simulink model "Simulation_cs_old"  (R2019a)
settings: Solver=ode5  StartTime=0.0  StopTime=inf  FixedStep=1/20  RelTol=1e-3
PreLoadFcn:
  | mbxruntime.callbacks.PreLoadFcn(bdroot);
PostLoadFcn:
  | mbxruntime.callbacks.PostLoadFcn(bdroot);
InitFcn:
  | mbxruntime.callbacks.InitFcn(bdroot);
StartFcn:
  | mbxruntime.callbacks.StartFcn(bdroot);
StopFcn:
  | mbxruntime.callbacks.StopFcn(bdroot);
model workspace: external: MAT-File .\Simulation_cs_hws.mat (data not in the file)
undefined symbols (not defined in the file or in its folder): DiscIntNeverNeededParam, InitImageOutputDir, mbxruntime, Simulation_cs_3ba1e87c6cdc7fd9, Simulation_cs_BMW_X5_SUV_1_Dynamics_Empty_STATE_BMW_X5_SUV_1_x0, Simulation_cs_BMW_X5_SUV_1_Dynamics_Empty_STATE_BMW_X5_SUV_1_y0, Simulation_cs_BMW_X5_SUV_1_Dynamics_Empty_STATE_BMW_X5_SUV_1_z0, Simulation_cs_dbe7801ee2d75073, Simulation_cs_f34d2d8469e03015
libraries: adeye_lib x45, robotlib x3, PreScanSimulinkLibrary x2, PreScanUsefulBlocks x1
(part 2 of 3)

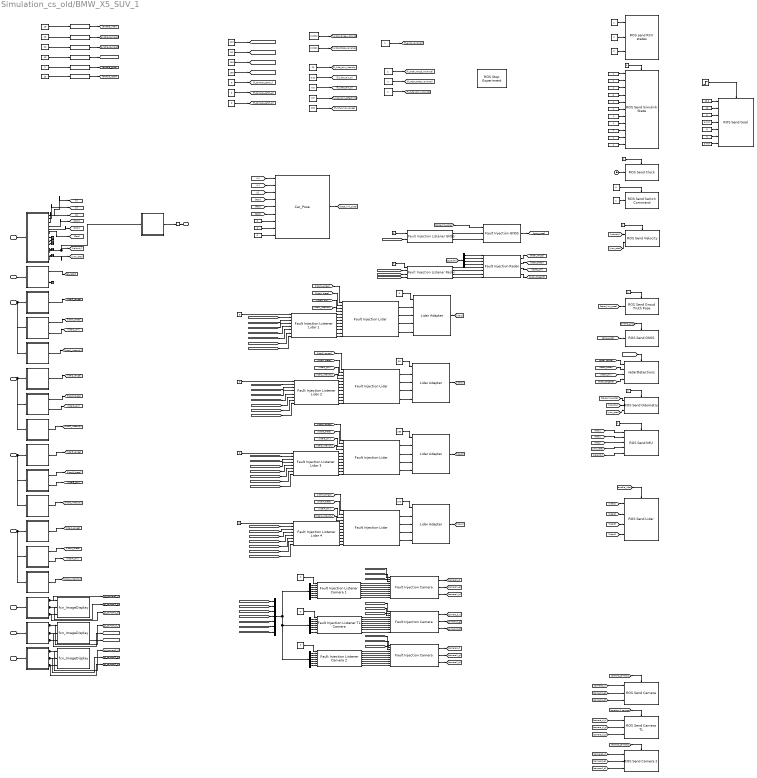
== system Simulation_cs_old/BMW_X5_SUV_1 ==
  note: CoG  compared
      | to the backwheels
      | center
  note: Lidar Fault injection Constants
  note: Radar Fault Injection Constants
  note: Rain model, Constants
  note: Camera Fault injection Constants
  note: GNSS Fault Injection Constants
  note: Gaussian random noise, Parameters
  note: Patch
  note: Frequencies at which the messages are sent
      |
      | For this send frequency to be respected, the simulink compilation sheet frequency
      | needs to be an integer multiple of this send frequency.
  SELF_BMW_X5_SUV_1 : Inport  Tag=inport/SelfPort  OutDataTypeStr=Bus: PRESCAN_SELFSENSORDATA  PortDimensions=1  SampleTime=1/20  BusOutputAsStruct=on
  Radar_1 : Inport  Tag=inport/Radar  Port=2  OutDataTypeStr=Bus: PRESCAN_SCANNERSENSOR_MESSAGE  PortDimensions=7  SampleTime=1/20  BusOutputAsStruct=on
  PointCloudSensor_1 : Inport  Tag=inport/PointCloudInport  Port=3  OutDataTypeStr=single  SampleTime=1/20  BusOutputAsStruct=on
  PointCloudSensor_2 : Inport  Tag=inport/PointCloudInport  Port=4  OutDataTypeStr=single  SampleTime=1/20  BusOutputAsStruct=on
  PointCloudSensor_3 : Inport  Tag=inport/PointCloudInport  Port=5  OutDataTypeStr=single  SampleTime=1/20  BusOutputAsStruct=on
  PointCloudSensor_4 : Inport  Tag=inport/PointCloudInport  Port=6  OutDataTypeStr=single  SampleTime=1/20  BusOutputAsStruct=on
  Camera_1 : Inport  Tag=inport/Camera/CameraSensor  Port=7  OutDataTypeStr=uint8  SampleTime=1/20  BusOutputAsStruct=on
  Camera_tl : Inport  Tag=inport/Camera/CameraSensor  Port=8  OutDataTypeStr=uint8  SampleTime=1/20  BusOutputAsStruct=on
  Camera_2 : Inport  Tag=inport/Camera/CameraSensor  Port=9  OutDataTypeStr=uint8  SampleTime=1/20  BusOutputAsStruct=on
  Activation request : Constant  OutDataTypeStr=Inherit: Inherit via back propagation
  Bus Selector1 : BusSelector  OutputSignals=Range[m],Theta[deg],Phi[deg],TargetTypeID[-]
  Camera_1_CM_Demux : Subsystem  Tag=demux/Camera/Color  mask{SensorName=Camera_1, hres=960, vres=720}
      mask prompts: SensorName "Sensor Name"; hres "Horizontal Resolution"; vres "Vertical Resolution"
      mask Help: eval('openHelp(457)')
      mask Display:
      | fprintf('MONO CAMERA:\n Color\n %s \n %d x %d px',SensorName,hres,vres)
      | port_label('output',1,'R')
      | port_label('output',2,'G')
      | port_label('output',3,'B')
  Camera_1_CM_Display : M-S-Function  Tag=CameraSensor_Color_Display  InitFcn=InitImageOutputDir(gcb);  FunctionName=fcn_ImageDisplay  Parameters=SensorName EnableDisplay EnablePosition DisplayPosition FigureHandle SaveResults BitmapFormat TempOutputDir CameraType DataType  mask(PreScan Color Display Block){SensorName=Camera_1, EnableDisplay=on, EnablePosition=off, DisplayPosition=[10 10 960 720], FigureHandle=15805, SaveResults=off, Format=PNG, TempOutputDir=0, CameraType=Mono, DataType=uint8}
      mask prompts: SensorName "User Specified: Title of Display"; EnableDisplay "Active"; EnablePosition "Set Display window position"; DisplayPosition "Display window position [xpos ypos width height]"; FigureHandle "Unique Handle"; SaveResults "Save results"; TempOutputDir "OutputDir"; CameraType "Camera Type"; DataType "Image Data Type"
      mask help: This block displays the RGB output of a PreScan camera sensor.
      mask init:
      | if EnableDisplay
      |     EnableString='';
      |     EnableColor='gray';
      | else
      |     EnableString='INACTIVE';
      |     EnableColor='red';
      | end
      | switch Format
      |     case 1
      |         BitmapFormat = 'png';
      |     case 2
      |         BitmapFormat = 'bmp';
      |     case 3
      |         BitmapFormat = 'jpg';
      | end 
      | if CameraType==1
      |     CameraTypeName='MONO';
      |     PortNumber=0;
      | else
      |     CameraTypeName='STEREO';
      |     PortNumber=3;
      | end
      settings: CopyFcn=CopyFcnDisplay  DeleteFcn=PreScanBlockDeleteFcn;  ModelCloseFcn=fcn_ImageDisplay_ModelCloseFcn
      mask Help: eval('openHelp(457)')
      mask Callback EnablePosition:
      | MV=get_param(gcb,'MaskVisibilities');
      | if strcmp(get_param(gcb,'EnablePosition'),'on')
      |     MV{4}='on';
      | else
      |     MV{4}='off';
      | end
      | set_param(gcb,'MaskVisibilities',MV);
      | clear MV;
      mask TypeOptions Format: PNG | BMP | JPG
      mask TypeOptions CameraType: Mono | Stereo
      mask TypeOptions DataType: uint8 | single
      mask Display:
      | color(EnableColor);
      | fprintf('%s\n DISPLAY:\n Color \n %s',EnableString,SensorName)
      | port_label('input',1,'R')
      | port_label('input',2,'G')
      | port_label('input',3,'B')
      | port_label('input',PortNumber+1,'R')
      | port_label('input',PortNumber+2,'G')
      | port_label('input',PortNumber+3,'B')
  Camera_2_CM_Demux : Subsystem  Tag=demux/Camera/Color  mask{SensorName=Camera_2, hres=960, vres=720}
      mask prompts: SensorName "Sensor Name"; hres "Horizontal Resolution"; vres "Vertical Resolution"
      mask Help: eval('openHelp(457)')
      mask Display:
      | fprintf('MONO CAMERA:\n Color\n %s \n %d x %d px',SensorName,hres,vres)
      | port_label('output',1,'R')
      | port_label('output',2,'G')
      | port_label('output',3,'B')
  Camera_2_CM_Display : M-S-Function  Tag=CameraSensor_Color_Display  InitFcn=InitImageOutputDir(gcb);  FunctionName=fcn_ImageDisplay  Parameters=SensorName EnableDisplay EnablePosition DisplayPosition FigureHandle SaveResults BitmapFormat TempOutputDir CameraType DataType  mask(PreScan Color Display Block){SensorName=Camera_2, EnableDisplay=on, EnablePosition=off, DisplayPosition=[10 10 960 720], FigureHandle=15807, SaveResults=off, Format=PNG, TempOutputDir=0, CameraType=Mono, DataType=uint8}
      mask prompts: SensorName "User Specified: Title of Display"; EnableDisplay "Active"; EnablePosition "Set Display window position"; DisplayPosition "Display window position [xpos ypos width height]"; FigureHandle "Unique Handle"; SaveResults "Save results"; TempOutputDir "OutputDir"; CameraType "Camera Type"; DataType "Image Data Type"
      mask help: This block displays the RGB output of a PreScan camera sensor.
      mask init: same as Simulation_cs_old/BMW_X5_SUV_1/Camera_1_CM_Display
      settings: CopyFcn=CopyFcnDisplay  DeleteFcn=PreScanBlockDeleteFcn;  ModelCloseFcn=fcn_ImageDisplay_ModelCloseFcn
      mask Help: eval('openHelp(457)')
      mask Callback EnablePosition:
      | MV=get_param(gcb,'MaskVisibilities');
      | if strcmp(get_param(gcb,'EnablePosition'),'on')
      |     MV{4}='on';
      | else
      |     MV{4}='off';
      | end
      | set_param(gcb,'MaskVisibilities',MV);
      | clear MV;
      mask TypeOptions Format: PNG | BMP | JPG
      mask TypeOptions CameraType: Mono | Stereo
      mask TypeOptions DataType: uint8 | single
      mask Display:
      | color(EnableColor);
      | fprintf('%s\n DISPLAY:\n Color \n %s',EnableString,SensorName)
      | port_label('input',1,'R')
      | port_label('input',2,'G')
      | port_label('input',3,'B')
      | port_label('input',PortNumber+1,'R')
      | port_label('input',PortNumber+2,'G')
      | port_label('input',PortNumber+3,'B')
  Camera_tl_CM_Demux : Subsystem  Tag=demux/Camera/Color  mask{SensorName=Camera_tl, hres=960, vres=720}
      mask prompts: SensorName "Sensor Name"; hres "Horizontal Resolution"; vres "Vertical Resolution"
      mask Help: eval('openHelp(457)')
      mask Display:
      | fprintf('MONO CAMERA:\n Color\n %s \n %d x %d px',SensorName,hres,vres)
      | port_label('output',1,'R')
      | port_label('output',2,'G')
      | port_label('output',3,'B')
  Camera_tl_CM_Display : M-S-Function  Tag=CameraSensor_Color_Display  InitFcn=InitImageOutputDir(gcb);  FunctionName=fcn_ImageDisplay  Parameters=SensorName EnableDisplay EnablePosition DisplayPosition FigureHandle SaveResults BitmapFormat TempOutputDir CameraType DataType  mask(PreScan Color Display Block){SensorName=Camera_tl, EnableDisplay=on, EnablePosition=off, DisplayPosition=[10 10 960 720], FigureHandle=15806, SaveResults=off, Format=PNG, TempOutputDir=0, CameraType=Mono, DataType=uint8}
      mask prompts: SensorName "User Specified: Title of Display"; EnableDisplay "Active"; EnablePosition "Set Display window position"; DisplayPosition "Display window position [xpos ypos width height]"; FigureHandle "Unique Handle"; SaveResults "Save results"; TempOutputDir "OutputDir"; CameraType "Camera Type"; DataType "Image Data Type"
      mask help: This block displays the RGB output of a PreScan camera sensor.
      mask init: same as Simulation_cs_old/BMW_X5_SUV_1/Camera_1_CM_Display
      settings: CopyFcn=CopyFcnDisplay  DeleteFcn=PreScanBlockDeleteFcn;  ModelCloseFcn=fcn_ImageDisplay_ModelCloseFcn
      mask Help: eval('openHelp(457)')
      mask Callback EnablePosition:
      | MV=get_param(gcb,'MaskVisibilities');
      | if strcmp(get_param(gcb,'EnablePosition'),'on')
      |     MV{4}='on';
      | else
      |     MV{4}='off';
      | end
      | set_param(gcb,'MaskVisibilities',MV);
      | clear MV;
      mask TypeOptions Format: PNG | BMP | JPG
      mask TypeOptions CameraType: Mono | Stereo
      mask TypeOptions DataType: uint8 | single
      mask Display:
      | color(EnableColor);
      | fprintf('%s\n DISPLAY:\n Color \n %s',EnableString,SensorName)
      | port_label('input',1,'R')
      | port_label('input',2,'G')
      | port_label('input',3,'B')
      | port_label('input',PortNumber+1,'R')
      | port_label('input',PortNumber+2,'G')
      | port_label('input',PortNumber+3,'B')
  Car_Pose : adeye_lib/Car_Pose  SystemSampleTime=-1
  Clock : Clock
  CoG offset x : Constant  Value=0
  CoG offset y : Constant  Value=0
  CoG offset z : Constant  Value=0
  Demux : Demux  Outputs=7
  Demux1 : Demux  Outputs=7
  Demux2 : Demux  Outputs=7
  Detection : Constant
  Dynamics_Empty : Subsystem  Tag=Dynamics_Empty
      mask Help: eval('openHelp(202)')
      mask Display: port_label('output', 1, 'State');text(0,0,' Empty\n')
  EnableSendClock : Constant  OutDataTypeStr=Inherit: Inherit via back propagation
  EnableSendFeatures : Constant  Value=0  OutDataTypeStr=Inherit: Inherit via back propagation
  EnableSendGroundTruthPose : Constant
  EnableSendIMU : Constant  OutDataTypeStr=Inherit: Inherit via back propagation
  EnableSendOdometry : Constant
  EnableSendSwitch : Constant  Value=0  OutDataTypeStr=Inherit: Inherit via back propagation  SampleTime=-1
  EnableSendVelocity : Constant  OutDataTypeStr=Inherit: Inherit via back propagation
  FakeLocalization : Constant
  Fault : Constant  Value=0  OutDataTypeStr=Inherit: Inherit via back propagation
  Fault Injection Camera : adeye_lib/Fault Injection Camera  idy=200  idx=100  x=100  y=150  R=0  G=0  B=0
  Fault Injection Camera1 : adeye_lib/Fault Injection Camera  idy=200  idx=100  x=100  y=150  R=0  G=0  B=0
  Fault Injection Camera2 : adeye_lib/Fault Injection Camera  idy=200  idx=100  x=100  y=150  R=0  G=0  B=0
  Fault Injection GNSS : adeye_lib/Fault Injection GNSS  SystemSampleTime=-1
  Fault Injection Lidar{,1..3} (4 alike) : adeye_lib/Fault Injection Lidar  p=225*16
  Fault Injection Listener Camera 1 : adeye_lib/Fault Injection Listener Camera 1  SystemSampleTime=-1
  Fault Injection Listener Camera 2 : adeye_lib/Fault Injection Listener Camera 2  SystemSampleTime=-1
  Fault Injection Listener GNSS : adeye_lib/Fault Injection Listener GNSS  SystemSampleTime=-1
  Fault Injection Listener Lidar 1 : adeye_lib/Fault Injection Listener Lidar 1  SystemSampleTime=-1
  Fault Injection Listener Lidar 2 : adeye_lib/Fault Injection Listener Lidar 2  SystemSampleTime=-1
  Fault Injection Listener Lidar 3 : adeye_lib/Fault Injection Listener Lidar 3  SystemSampleTime=-1
  Fault Injection Listener Lidar 4 : adeye_lib/Fault Injection Listener Lidar 4  SystemSampleTime=-1
  Fault Injection Listener Radar : adeye_lib/Fault Injection Listener Radar  SystemSampleTime=-1
  Fault Injection Listener TL Camera : adeye_lib/Fault Injection Listener TL Camera  SystemSampleTime=-1
  Fault Injection Radar : adeye_lib/Fault Injection Radar  n=7
  FaultInjectionCamera1 : Constant  Value=0
  FaultInjectionCamera2 : Constant  Value=0
  FaultInjectionGNSS : Constant  Value=0  OutDataTypeStr=Inherit: Inherit via back propagation  SampleTime=0.05
  FaultInjectionLidar{1..4} (4 alike) : Constant  Value=0  OutDataTypeStr=Inherit: Inherit via back propagation
  FaultInjectionRadar : Constant  Value=0
  FaultInjectionTLCamera : Constant  Value=0
  GoalOrientW : Constant  Value=0.707
  GoalOrientX : Constant  Value=0
  GoalOrientY : Constant  Value=0
  GoalOrientZ : Constant  Value=0.707
  GoalPoseX : Constant  Value=23.3
  GoalPoseY : Constant  Value=40
  GoalPoseZ : Constant  Value=0
  Initial checks : Constant  OutDataTypeStr=Inherit: Inherit via back propagation
  Lidar Adapter{,1..3} (4 alike) : adeye_lib/Lidar Adapter  SystemSampleTime=-1
  Localization : Constant  Value=0
  Map : Constant
  MissionPlanning : Constant
  MotionPlanning : Constant
  Mux : Mux  Inputs=7
  OrientationLidar1 : Constant  Value=0  OutDataTypeStr=Inherit: Inherit via back propagation
  OrientationLidar2 : Constant  Value=90  OutDataTypeStr=Inherit: Inherit via back propagation
  OrientationLidar3 : Constant  Value=180  OutDataTypeStr=Inherit: Inherit via back propagation
  OrientationLidar4 : Constant  Value=270  OutDataTypeStr=Inherit: Inherit via back propagation
  PointCloudSensor_1_Angles_Demux : Subsystem  Tag=demux/PCS/Angles  mask{SensorName=PointCloudSensor_1, offset=225, hres=225, vres=16}
      mask prompts: SensorName "Sensor Name"; offset "Data Start"; hres "Horizontal Resolution"; vres "Vertical Resolution"
      mask Help: eval('openHelp(6400)')
      mask Display:
      | fprintf('Point Cloud:\n Data\n %s \n %d x %d px',SensorName,hres,vres)
      | port_label('output',1,'Theta')
      | port_label('output',2,'Phi')
  PointCloudSensor_1_Intensity_Demux : Subsystem  Tag=demux/PCS/Intensity  mask{SensorName=PointCloudSensor_1, offset=675, hres=225, vres=16}
      mask prompts: SensorName "Sensor Name"; offset "Data Start"; hres "Horizontal Resolution"; vres "Vertical Resolution"
      mask Help: eval('openHelp(6400)')
      mask Display:
      | fprintf('Point Cloud:\n Data\n %s \n %d x %d px',SensorName,hres,vres)
      | port_label('output',1,'Intensity')
  PointCloudSensor_1_Range_Demux : Subsystem  Tag=demux/PCS/Range  mask{SensorName=PointCloudSensor_1, offset=0, hres=225, vres=16}
      mask prompts: SensorName "Sensor Name"; offset "Data Start"; hres "Horizontal Resolution"; vres "Vertical Resolution"
      mask Help: eval('openHelp(6400)')
      mask Display:
      | fprintf('Point Cloud:\n Data\n %s \n %d x %d px',SensorName,hres,vres)
      | port_label('output',1,'Range')
  PointCloudSensor_2_Angles_Demux : Subsystem  Tag=demux/PCS/Angles  mask{SensorName=PointCloudSensor_2, offset=225, hres=225, vres=16}
      mask prompts: SensorName "Sensor Name"; offset "Data Start"; hres "Horizontal Resolution"; vres "Vertical Resolution"
      mask Help: eval('openHelp(6400)')
      mask Display:
      | fprintf('Point Cloud:\n Data\n %s \n %d x %d px',SensorName,hres,vres)
      | port_label('output',1,'Theta')
      | port_label('output',2,'Phi')
  PointCloudSensor_2_Intensity_Demux : Subsystem  Tag=demux/PCS/Intensity  mask{SensorName=PointCloudSensor_2, offset=675, hres=225, vres=16}
      mask prompts: SensorName "Sensor Name"; offset "Data Start"; hres "Horizontal Resolution"; vres "Vertical Resolution"
      mask Help: eval('openHelp(6400)')
      mask Display:
      | fprintf('Point Cloud:\n Data\n %s \n %d x %d px',SensorName,hres,vres)
      | port_label('output',1,'Intensity')
  PointCloudSensor_2_Range_Demux : Subsystem  Tag=demux/PCS/Range  mask{SensorName=PointCloudSensor_2, offset=0, hres=225, vres=16}
      mask prompts: SensorName "Sensor Name"; offset "Data Start"; hres "Horizontal Resolution"; vres "Vertical Resolution"
      mask Help: eval('openHelp(6400)')
      mask Display:
      | fprintf('Point Cloud:\n Data\n %s \n %d x %d px',SensorName,hres,vres)
      | port_label('output',1,'Range')
  PointCloudSensor_3_Angles_Demux : Subsystem  Tag=demux/PCS/Angles  mask{SensorName=PointCloudSensor_3, offset=225, hres=225, vres=16}
      mask prompts: SensorName "Sensor Name"; offset "Data Start"; hres "Horizontal Resolution"; vres "Vertical Resolution"
      mask Help: eval('openHelp(6400)')
      mask Display:
      | fprintf('Point Cloud:\n Data\n %s \n %d x %d px',SensorName,hres,vres)
      | port_label('output',1,'Theta')
      | port_label('output',2,'Phi')
  PointCloudSensor_3_Intensity_Demux : Subsystem  Tag=demux/PCS/Intensity  mask{SensorName=PointCloudSensor_3, offset=675, hres=225, vres=16}
      mask prompts: SensorName "Sensor Name"; offset "Data Start"; hres "Horizontal Resolution"; vres "Vertical Resolution"
      mask Help: eval('openHelp(6400)')
      mask Display:
      | fprintf('Point Cloud:\n Data\n %s \n %d x %d px',SensorName,hres,vres)
      | port_label('output',1,'Intensity')
  PointCloudSensor_3_Range_Demux : Subsystem  Tag=demux/PCS/Range  mask{SensorName=PointCloudSensor_3, offset=0, hres=225, vres=16}
      mask prompts: SensorName "Sensor Name"; offset "Data Start"; hres "Horizontal Resolution"; vres "Vertical Resolution"
      mask Help: eval('openHelp(6400)')
      mask Display:
      | fprintf('Point Cloud:\n Data\n %s \n %d x %d px',SensorName,hres,vres)
      | port_label('output',1,'Range')
  PointCloudSensor_4_Angles_Demux : Subsystem  Tag=demux/PCS/Angles  mask{SensorName=PointCloudSensor_4, offset=225, hres=225, vres=16}
      mask prompts: SensorName "Sensor Name"; offset "Data Start"; hres "Horizontal Resolution"; vres "Vertical Resolution"
      mask Help: eval('openHelp(6400)')
      mask Display:
      | fprintf('Point Cloud:\n Data\n %s \n %d x %d px',SensorName,hres,vres)
      | port_label('output',1,'Theta')
      | port_label('output',2,'Phi')
  PointCloudSensor_4_Intensity_Demux : Subsystem  Tag=demux/PCS/Intensity  mask{SensorName=PointCloudSensor_4, offset=675, hres=225, vres=16}
      mask prompts: SensorName "Sensor Name"; offset "Data Start"; hres "Horizontal Resolution"; vres "Vertical Resolution"
      mask Help: eval('openHelp(6400)')
      mask Display:
      | fprintf('Point Cloud:\n Data\n %s \n %d x %d px',SensorName,hres,vres)
      | port_label('output',1,'Intensity')
  PointCloudSensor_4_Range_Demux : Subsystem  Tag=demux/PCS/Range  mask{SensorName=PointCloudSensor_4, offset=0, hres=225, vres=16}
      mask prompts: SensorName "Sensor Name"; offset "Data Start"; hres "Horizontal Resolution"; vres "Vertical Resolution"
      mask Help: eval('openHelp(6400)')
      mask Display:
      | fprintf('Point Cloud:\n Data\n %s \n %d x %d px',SensorName,hres,vres)
      | port_label('output',1,'Range')
  ROS Send Camera : adeye_lib/ROS Send Camera  SystemSampleTime=-1
  ROS Send Camera 2 : adeye_lib/ROS Send Camera 2  SystemSampleTime=-1
  ROS Send Camera TL : adeye_lib/ROS Send Camera TL  SystemSampleTime=-1
  ROS Send Clock : adeye_lib/ROS Send Clock  Priority=1  SystemSampleTime=-1
  ROS Send GNSS : adeye_lib/ROS Send GNSS  SystemSampleTime=-1
  ROS Send Goal : adeye_lib/ROS Send Goal  SystemSampleTime=-1
  ROS Send Groud Truth Pose : adeye_lib/ROS Send Groud Truth Pose  SystemSampleTime=-1
  ROS Send IMU : adeye_lib/ROS Send IMU  SystemSampleTime=-1
  ROS Send Lidar : adeye_lib/ROS Send Lidar  SystemSampleTime=-1
  ROS Send Odometry : adeye_lib/ROS Send Odometry  SystemSampleTime=-1
  ROS Send Simulink State : adeye_lib/ROS Send Simulink State  SystemSampleTime=-1
  ROS Send Switch Command : adeye_lib/ROS Send Switch Command  SystemSampleTime=-1
  ROS Send Velocity : adeye_lib/ROS Send Velocity  SystemSampleTime=-1
  "ROS Stop Experiment " : adeye_lib/ROS Stop Experiment  SystemSampleTime=-1
  ROS send RCV states : adeye_lib/ROS send RCV states  SystemSampleTime=-1
  Radar_1_Demux : Subsystem  Tag=demux/Radar  TreatAsAtomicUnit=on  mask(PreScan Demux Block: Radar){MAXMESSAGES=7}
      mask prompts: MAXMESSAGES "Number of Objects"
      mask help:
      | The Radar Sensor is a detailed sensor based on a physical radar
      | model that includes Antenna GAIN Maps (AGM) and atmospheric
      | attenuation.
      |
      | For more information, please click Help.
      mask Help: eval('openHelp(1464)')
      mask Display:
      | port_label('input',1,'Radar')
      | port_label('output',1,'Radar Data')
      | port_label('output',2,'Timestamp [s]')
  Recording : Constant
  Rviz : Constant
  SELF_Demux : Subsystem  Tag=demux/SelfPort  mask(PreScan Demux Block:){}
      mask help:
      | The SELF port shows (state) information of the actor itself. The outputs are position in the experiment's axis system and the GPS coordinates, and the object's absolute velocity and compass heading.
      |
      | For more information, please click Help.
      settings: DeleteFcn=PreScanBlockDeleteFcn;
      mask Help: eval('openHelp(462)')
      mask Display:
      | port_label('output',1,'x [m]')
      | port_label('output',2,'y [m]')
      | port_label('output',3,'z [m]','texmode','on')
      | port_label('output',4,'Rotx [deg]','texmode','on')
      | port_label('output',5,'Roty [deg]','texmode','on')
      | port_label('output',6,'Rotz [deg]','texmode','on')
      | port_label('output',7,'GPS lat [deg]','texmode','on')
      | port_label('output',8,'GPS long [deg]','texmode','on')
      | port_label('output',9,'GPS alt [m]','texmode','on')
      | port_label('output',10,'Velocity [m/s]')
      | port_label('output',11,'Heading [deg]')
      | port_label('output',12,'Yaw rate [deg/s]')
      | port_label('output',13,'Timestamp [s]')
  STATE_BMW_X5_SUV_1_rc : RateTransition  Tag=mux_rc/StatePort  OutPortSampleTimeOpt=Inherit
  Sensing : Constant
  Ssmp : Constant
  Step : Step  Time=5  Before=1  After=0  SampleTime=0  VectorParams1D=off
  Switch : Constant
  SwitchCommand : Constant  OutDataTypeStr=Inherit: Inherit via back propagation  SampleTime=-1
  Terminator_{1..6} (6 alike) : Terminator
  fi_camera_patch_b : Constant  Value=0
  fi_camera_patch_g : Constant  Value=0
  fi_camera_patch_r : Constant  Value=0
  fi_camera_patch_size_x : Constant  Value=100
  fi_camera_patch_size_y : Constant  Value=100
  fi_camera_patch_start_x : Constant  Value=110
  fi_camera_patch_start_y : Constant  Value=50
  fi_gnss_variance : Constant
  fi_lidar_max_range : Constant  Value=150
  fi_lidar_rain_a : Constant  Value=0.01
  fi_lidar_rain_b : Constant  Value=0.6
  fi_lidar_rain_intensity : Constant  Value=20
  fi_lidar_rain_reflectivity : Constant  Value=0.9
  fi_lidar_range_variance : Constant  Value=0.0001
  fi_lidar_theta_variance : Constant  Value=0.0001
  fi_radar_phi_variance : Constant
  fi_radar_range_variance : Constant
  fi_radar_theta_variance : Constant
  frequency_evaluator_camera1 : adeye_lib/frequency_evaluator  SystemSampleTime=-1
  frequency_evaluator_camera2 : adeye_lib/frequency_evaluator  SystemSampleTime=-1
  frequency_evaluator_gnss : adeye_lib/frequency_evaluator  SystemSampleTime=-1
  frequency_evaluator_lidar : adeye_lib/frequency_evaluator  SystemSampleTime=-1
      link override Constant: Value=0.999
  frequency_evaluator_radar : adeye_lib/frequency_evaluator  SystemSampleTime=-1
  frequency_evaluator_tl_camera : adeye_lib/frequency_evaluator  SystemSampleTime=-1
  radarDetections : adeye_lib/radarDetections  SystemSampleTime=-1
  send_frequency_camera1 : Constant  Value=20
  send_frequency_camera2 : Constant  Value=20
  send_frequency_gnss : Constant
  send_frequency_lidar : Constant  Value=10
  send_frequency_radar : Constant  Value=20
  send_frequency_tl_camera : Constant  Value=10
  STATE_BMW_X5_SUV_1_bus : Outport  Tag=outport/StatePort  OutDataTypeStr=Bus: PRESCAN_STATEACTUATORDATA  PortDimensions=1  SampleTime=1/20
  wires:
  Fault Injection Lidar1/3 -> Lidar Adapter1/4
  [lidar2] -> ROS Send Lidar/2
  fi_camera_patch_r/1 -> [fi_camera_patch_r]
  fi_radar_range_variance/1 -> [fi_radar_range_variance]
  fi_lidar_range_variance/1 -> [fi_lidar_range_variance]
  [enable_gnss] -> ROS Send GNSS/Enable
  [x] -> Car_Pose/1
  EnableSendClock/1 -> ROS Send Clock/Enable
  [fi_lidar_rain_intensity] -> Fault Injection Listener Lidar 4/4
  send_frequency_lidar/1 -> frequency_evaluator_lidar/1
  fi_camera_patch_size_y/1 -> [fi_camera_patch_size_y]
  Initial checks/1 -> ROS send RCV states/1
  [lidar4_intensity] -> Fault Injection Lidar3/4
  fi_camera_patch_start_y/1 -> [fi_camera_patch_start_y]
  [gt_radar] -> Bus Selector1/1
  fi_camera_patch_size_x/1 -> [fi_camera_patch_size_x]
  fi_radar_theta_variance/1 -> [fi_radar_theta_variance]
  fi_lidar_rain_reflectivity/1 -> [fi_lidar_rain_reflectivity]
  [enable_radar] -> radarDetections/Enable
  fi_lidar_rain_intensity/1 -> [fi_lidar_rain_intensity]
  send_frequency_camera2/1 -> frequency_evaluator_camera2/1
  Fault Injection Listener Lidar 4/8 -> Fault Injection Lidar3/12
  GoalOrientW/1 -> ROS Send Goal/4
  OrientationLidar1/1 -> Lidar Adapter/1
  [radar_targetID] -> radarDetections/4
  fi_gnss_variance/1 -> [fi_gnss_variance]
  Demux1/6 -> Fault Injection Listener TL Camera/7
  frequency_evaluator_gnss/1 -> [enable_gnss]
  [lidar2_intensity] -> Fault Injection Lidar1/4
  Fault Injection Listener Camera 2/5 -> Fault Injection Camera/8
  frequency_evaluator_camera2/1 -> [enable_camera2]
  Demux/6 -> Fault Injection Listener Camera 1/7
  GoalOrientY/1 -> ROS Send Goal/6
  Fault Injection Listener Lidar 1/7 -> Fault Injection Lidar/11
  [lidar4_theta] -> Fault Injection Lidar3/2
  Camera_tl_CM_Demux/3(B) -> [gt_camera_tl_b], Camera_tl_CM_Display/3
  frequency_evaluator_radar/1 -> [enable_radar]
  [fi_lidar_rain_b] -> Fault Injection Listener Lidar 3/6
  [gnss_pose] -> ROS Send GNSS/1
  EnableSendOdometry/1 -> ROS Send Odometry/Enable
  EnableSendGroundTruthPose/1 -> ROS Send Groud Truth Pose/Enable
  [enable_lidar] -> ROS Send Lidar/Enable
  Fault Injection Listener Radar/1 -> Fault Injection Radar/5
  [velocity] -> ROS Send Velocity/1
  Switch/1 -> ROS Send Simulink State/9
  GoalPoseX/1 -> ROS Send Goal/1
  Fault Injection Listener TL Camera/1 -> Fault Injection Camera2/4
  Ssmp/1 -> ROS Send Simulink State/10
  Fault Injection Listener Camera 1/7 -> Fault Injection Camera1/10
  Camera_tl_CM_Demux/1(R) -> [gt_camera_tl_r], Camera_tl_CM_Display/1
  Camera_1_CM_Demux/2(G) -> [gt_camera1_g], Camera_1_CM_Display/2
  Fault Injection Listener Lidar 3/5 -> Fault Injection Lidar2/9
  Camera_2_CM_Demux/1(R) -> [gt_camera2_r], Camera_2_CM_Display/1
  Camera_tl_CM_Demux/2(G) -> [gt_camera_tl_g], Camera_tl_CM_Display/2
  [camera2_r] -> ROS Send Camera 2/1
  [camera_tl_r] -> ROS Send Camera TL/1
  Localization/1 -> ROS Send Simulink State/4
  Fault Injection Camera2/3 -> [camera_tl_b]
  Fault Injection Listener Lidar 1/5 -> Fault Injection Lidar/9
  [lidar4] -> ROS Send Lidar/4
  FaultInjectionGNSS/1 -> Fault Injection Listener GNSS/1
  Demux1/2 -> Fault Injection Listener TL Camera/3
  Rviz/1 -> ROS Send Simulink State/11
  fi_lidar_theta_variance/1 -> [fi_lidar_theta_variance]
  Fault Injection Listener Lidar 2/2 -> Fault Injection Lidar1/6
  fi_radar_phi_variance/1 -> [fi_radar_phi_variance]
  Fault Injection Listener Lidar 4/7 -> Fault Injection Lidar3/11
  [fi_radar_phi_variance] -> Fault Injection Listener Radar/4
  GoalPoseY/1 -> ROS Send Goal/2
  Car_Pose/1 -> [base_link_pose]
  Fault Injection Camera/1 -> [camera2_r]
  fi_camera_patch_start_x/1 -> [fi_camera_patch_start_x]
  Bus Selector1/1 -> Fault Injection Radar/1  "<Range[m]>"
  [fi_lidar_rain_b] -> Fault Injection Listener Lidar 2/6
  [fi_lidar_rain_b] -> Fault Injection Listener Lidar 4/6
  [fi_gnss_variance] -> Fault Injection Listener GNSS/2
  [fi_lidar_rain_a] -> Fault Injection Listener Lidar 4/5
  send_frequency_camera1/1 -> frequency_evaluator_camera1/1
  FaultInjectionCamera2/1 -> Fault Injection Listener Camera 2/1
  [gt_camera2_b] -> Fault Injection Camera/3
  Fault Injection Listener Lidar 3/7 -> Fault Injection Lidar2/11
  [fi_lidar_rain_reflectivity] -> Fault Injection Listener Lidar 2/7
  Demux/4 -> Fault Injection Listener Camera 1/5
  frequency_evaluator_lidar/1 -> [enable_lidar]
  Fault Injection Listener Lidar 4/6 -> Fault Injection Lidar3/10
  [lidar3_intensity] -> Fault Injection Lidar2/4
  frequency_evaluator_tl_camera/1 -> [enable_tl_camera]
  Fault Injection Listener TL Camera/8 -> Fault Injection Camera2/11
  [fi_lidar_rain_intensity] -> Fault Injection Listener Lidar 2/4
  [enable_camera2] -> ROS Send Camera 2/Enable
  Fault Injection Lidar1/1 -> Lidar Adapter1/2
  FaultInjectionLidar2/1 -> Fault Injection Listener Lidar 2/1
  Fault Injection Listener Camera 1/6 -> Fault Injection Camera1/9
  Fault Injection Camera1/1 -> [camera1_r]
  Fault Injection Listener Lidar 3/2 -> Fault Injection Lidar2/6
  [lidar3_phi] -> Fault Injection Lidar2/3
  [yaw_rate] -> ROS Send Velocity/2
  Fault Injection Listener Lidar 4/5 -> Fault Injection Lidar3/9
  Fault/1 -> ROS send RCV states/3
  Demux2/5 -> Fault Injection Listener Camera 2/6
  Fault Injection Listener Lidar 3/6 -> Fault Injection Lidar2/10
  Fault Injection Lidar1/2 -> Lidar Adapter1/3
  Fault Injection Listener Lidar 4/1 -> Fault Injection Lidar3/5
  fi_lidar_max_range/1 -> [fi_lidar_max_range]
  [lidar2_range] -> Fault Injection Lidar1/1
  Fault Injection Listener Lidar 4/4 -> Fault Injection Lidar3/8
  Demux/5 -> Fault Injection Listener Camera 1/6
  Fault Injection Lidar3/3 -> Lidar Adapter3/4
  Fault Injection Listener Lidar 2/5 -> Fault Injection Lidar1/9
  Fault Injection Camera1/2 -> [camera1_g]
  [fi_camera_patch_size_x] -> Mux/3
  [fi_lidar_max_range] -> Fault Injection Listener Lidar 3/8
  [radar_theta] -> radarDetections/2
  [Rotx] -> Car_Pose/4
  [base_link_pose] -> ROS Send Groud Truth Pose/1
  Fault Injection Camera/3 -> [camera2_b]
  [enable_tl_camera] -> ROS Send Camera TL/Enable
  GoalOrientX/1 -> ROS Send Goal/5
  Fault Injection Listener Camera 2/3 -> Fault Injection Camera/6
  Lidar Adapter1/1 -> [lidar2]
  Detection/1 -> ROS Send Simulink State/6
  [fi_camera_patch_g] -> Mux/6
  [lidar1_theta] -> Fault Injection Lidar/2
  [fi_lidar_max_range] -> Fault Injection Listener Lidar 2/8
  EnableSendIMU/1 -> ROS Send IMU/Enable
  [camera1_g] -> ROS Send Camera/2
  [fi_lidar_rain_a] -> Fault Injection Listener Lidar 1/5
  GoalOrientZ/1 -> ROS Send Goal/7
  Demux/7 -> Fault Injection Listener Camera 1/8
  [lidar3] -> ROS Send Lidar/3
  [velocity] -> ROS Send Odometry/2
  [yaw_rate] -> ROS Send IMU/4
  [fi_lidar_rain_reflectivity] -> Fault Injection Listener Lidar 3/7
  [Rotx] -> ROS Send IMU/1
  Fault Injection Lidar2/2 -> Lidar Adapter2/3
  [fi_lidar_rain_intensity] -> Fault Injection Listener Lidar 3/4
  [gt_camera_tl_g] -> Fault Injection Camera2/2
  [fi_radar_range_variance] -> Fault Injection Listener Radar/2
  Fault Injection Lidar3/1 -> Lidar Adapter3/2
  Sensing/1 -> ROS Send Simulink State/3
  [camera2_b] -> ROS Send Camera 2/3
  SwitchCommand/1 -> ROS Send Switch Command/1
  Camera_1_CM_Demux/1(R) -> [gt_camera1_r], Camera_1_CM_Display/1
  Fault Injection Listener Lidar 4/3 -> Fault Injection Lidar3/7
  [yaw_rate] -> ROS Send Odometry/3
  [radar_range] -> radarDetections/1
  [lidar2_theta] -> Fault Injection Lidar1/2
  Fault Injection Listener Lidar 2/4 -> Fault Injection Lidar1/8
  Fault Injection Listener Lidar 2/1 -> Fault Injection Lidar1/5
  [fi_lidar_max_range] -> Fault Injection Listener Lidar 4/8
  FaultInjectionRadar/1 -> Fault Injection Listener Radar/1
  [fi_lidar_theta_variance] -> Fault Injection Listener Lidar 1/3
  [lidar1] -> ROS Send Lidar/1
  [camera1_b] -> ROS Send Camera/3
  [fi_camera_patch_b] -> Mux/7
  Clock/1 -> ROS Send Clock/1
  Fault Injection Listener TL Camera/5 -> Fault Injection Camera2/8
  FaultInjectionLidar3/1 -> Fault Injection Listener Lidar 3/1
  Mux/1 -> Demux/1, Demux1/1, Demux2/1
  [enable_camera1] -> ROS Send Camera/Enable
  EnableSendSwitch/1 -> ROS Send Switch Command/Enable
  Fault Injection Listener Camera 1/4 -> Fault Injection Camera1/7
  MissionPlanning/1 -> ROS Send Simulink State/7
  Fault Injection Listener Lidar 1/8 -> Fault Injection Lidar/12
  Fault Injection Radar/3 -> [radar_phi]
  Fault Injection Listener Camera 2/6 -> Fault Injection Camera/9
  [Roty] -> ROS Send IMU/2
  [fi_camera_patch_start_x] -> Mux/1
  fi_camera_patch_b/1 -> [fi_camera_patch_b]
  Step/1 -> ROS Send Goal/Enable
  Fault Injection Listener Camera 2/8 -> Fault Injection Camera/11
  Fault Injection Lidar/1 -> Lidar Adapter/2
  Camera_2_CM_Demux/3(B) -> [gt_camera2_b], Camera_2_CM_Display/3
  Demux2/1 -> Fault Injection Listener Camera 2/2
  Fault Injection Camera2/2 -> [camera_tl_g]
  fi_lidar_rain_b/1 -> [fi_lidar_rain_b]
  [fi_radar_theta_variance] -> Fault Injection Listener Radar/3
  CoG offset x/1 -> Car_Pose/7
  [fi_lidar_max_range] -> Fault Injection Listener Lidar 1/8
  Fault Injection Radar/2 -> [radar_theta]
  Demux/1 -> Fault Injection Listener Camera 1/2
  Demux2/6 -> Fault Injection Listener Camera 2/7
  Demux1/5 -> Fault Injection Listener TL Camera/6
  [velocity] -> ROS Send IMU/5
  [gt_camera1_r] -> Fault Injection Camera1/1
  Fault Injection Listener TL Camera/4 -> Fault Injection Camera2/7
  CoG offset y/1 -> Car_Pose/8
  Recording/1 -> ROS Send Simulink State/1
  [fi_lidar_rain_b] -> Fault Injection Listener Lidar 1/6
  [Roty] -> Car_Pose/5
  [gt_camera1_b] -> Fault Injection Camera1/3
  Bus Selector1/4 -> Fault Injection Radar/4  "<TargetTypeID[-]>"
  Fault Injection Listener Lidar 3/1 -> Fault Injection Lidar2/5
  Fault Injection Lidar2/4 -> Lidar Adapter2/5
  [Rotz] -> Car_Pose/6
  Activation request/1 -> ROS send RCV states/2
  Fault Injection Lidar2/3 -> Lidar Adapter2/4
  [gt_camera2_r] -> Fault Injection Camera/1
  FaultInjectionCamera1/1 -> Fault Injection Listener Camera 1/1
  Fault Injection Listener Camera 1/3 -> Fault Injection Camera1/6
  fi_lidar_rain_a/1 -> [fi_lidar_rain_a]
  Demux/2 -> Fault Injection Listener Camera 1/3
  [base_link_pose] -> ROS Send Odometry/1
  [fi_lidar_range_variance] -> Fault Injection Listener Lidar 3/2
  Fault Injection Lidar3/4 -> Lidar Adapter3/5
  [radar_phi] -> radarDetections/3
  Fault Injection Listener Lidar 2/7 -> Fault Injection Lidar1/11
  FaultInjectionTLCamera/1 -> Fault Injection Listener TL Camera/1
  Demux/3 -> Fault Injection Listener Camera 1/4
  [fi_lidar_rain_reflectivity] -> Fault Injection Listener Lidar 4/7
  [fi_lidar_range_variance] -> Fault Injection Listener Lidar 4/2
  SELF_Demux/1(x [m]) -> [x]
  [fi_lidar_rain_reflectivity] -> Fault Injection Listener Lidar 1/7
  FakeLocalization/1 -> ROS Send Simulink State/5
  [lidar4_range] -> Fault Injection Lidar3/1
  Fault Injection Listener Camera 1/5 -> Fault Injection Camera1/8
  [fi_camera_patch_r] -> Mux/5
  EnableSendFeatures/1 -> ROS Send Simulink State/Enable
  Fault Injection Listener TL Camera/3 -> Fault Injection Camera2/6
  Fault Injection Listener Radar/3 -> Fault Injection Radar/7
  Fault Injection Listener Lidar 1/2 -> Fault Injection Lidar/6
  Fault Injection Listener Camera 2/7 -> Fault Injection Camera/10
  [gt_camera_tl_r] -> Fault Injection Camera2/1
  GoalPoseZ/1 -> ROS Send Goal/3
  Fault Injection Camera/2 -> [camera2_g]
  Demux1/3 -> Fault Injection Listener TL Camera/4
  Fault Injection Listener Camera 1/8 -> Fault Injection Camera1/11
  Fault Injection Listener GNSS/1 -> Fault Injection GNSS/2
  Fault Injection Listener Lidar 1/4 -> Fault Injection Lidar/8
  Fault Injection Listener GNSS/2 -> Fault Injection GNSS/3
  [gt_camera2_g] -> Fault Injection Camera/2
  FaultInjectionLidar1/1 -> Fault Injection Listener Lidar 1/1
  frequency_evaluator_camera1/1 -> [enable_camera1]
  [Rotz] -> ROS Send IMU/3
  Fault Injection Radar/4 -> [radar_targetID]
  [fi_lidar_rain_intensity] -> Fault Injection Listener Lidar 1/4
  [fi_camera_patch_size_y] -> Mux/4
  fi_camera_patch_g/1 -> [fi_camera_patch_g]
  Fault Injection Listener Lidar 3/4 -> Fault Injection Lidar2/8
  FaultInjectionLidar4/1 -> Fault Injection Listener Lidar 4/1
  Map/1 -> ROS Send Simulink State/2
  [fi_lidar_rain_a] -> Fault Injection Listener Lidar 3/5
  Lidar Adapter/1 -> [lidar1]
  send_frequency_radar/1 -> frequency_evaluator_radar/1
  Bus Selector1/2 -> Fault Injection Radar/2  "<Theta[deg]>"
  [fi_lidar_rain_a] -> Fault Injection Listener Lidar 2/5
  Fault Injection Listener Radar/4 -> Fault Injection Radar/8
  Fault Injection Listener Camera 2/2 -> Fault Injection Camera/5
  Bus Selector1/3 -> Fault Injection Radar/3  "<Phi[deg]>"
  Fault Injection Listener Radar/2 -> Fault Injection Radar/6
  send_frequency_tl_camera/1 -> frequency_evaluator_tl_camera/1
  Fault Injection Listener Lidar 1/1 -> Fault Injection Lidar/5
  [lidar2_phi] -> Fault Injection Lidar1/3
  Fault Injection Listener Camera 1/2 -> Fault Injection Camera1/5
  Demux1/4 -> Fault Injection Listener TL Camera/5
  [base_link_pose] -> Fault Injection GNSS/1
  Camera_2_CM_Demux/2(G) -> [gt_camera2_g], Camera_2_CM_Display/2
  OrientationLidar2/1 -> Lidar Adapter1/1
  EnableSendVelocity/1 -> ROS Send Velocity/Enable
  Fault Injection GNSS/1 -> [gnss_pose]
  send_frequency_gnss/1 -> frequency_evaluator_gnss/1
  Fault Injection Listener Lidar 1/3 -> Fault Injection Lidar/7
  Fault Injection Listener TL Camera/6 -> Fault Injection Camera2/9
  Demux2/4 -> Fault Injection Listener Camera 2/5
  OrientationLidar3/1 -> Lidar Adapter2/1
  Fault Injection Camera2/1 -> [camera_tl_r]
  [fi_camera_patch_start_y] -> Mux/2
  [fi_lidar_theta_variance] -> Fault Injection Listener Lidar 2/3
  Fault Injection Listener Lidar 3/8 -> Fault Injection Lidar2/12
  Fault Injection Listener Camera 2/4 -> Fault Injection Camera/7
  Demux2/7 -> Fault Injection Listener Camera 2/8
  Demux2/3 -> Fault Injection Listener Camera 2/4
  [fi_lidar_theta_variance] -> Fault Injection Listener Lidar 3/3
  [gt_camera_tl_b] -> Fault Injection Camera2/3
  Fault Injection Listener Lidar 2/6 -> Fault Injection Lidar1/10
  [lidar1_range] -> Fault Injection Lidar/1
  MotionPlanning/1 -> ROS Send Simulink State/8
  Lidar Adapter3/1 -> [lidar4]
  Fault Injection Lidar/4 -> Lidar Adapter/5
  Fault Injection Radar/1 -> [radar_range]
  OrientationLidar4/1 -> Lidar Adapter3/1
  [z] -> Car_Pose/3
  [fi_lidar_range_variance] -> Fault Injection Listener Lidar 1/2
  Fault Injection Listener Lidar 2/3 -> Fault Injection Lidar1/7
  Demux1/1 -> Fault Injection Listener TL Camera/2
  [y] -> Car_Pose/2
  Fault Injection Listener TL Camera/2 -> Fault Injection Camera2/5
  Fault Injection Lidar/3 -> Lidar Adapter/4
  [camera_tl_b] -> ROS Send Camera TL/3
  Fault Injection Lidar2/1 -> Lidar Adapter2/2
  [lidar1_phi] -> Fault Injection Lidar/3
  Fault Injection Listener Lidar 3/3 -> Fault Injection Lidar2/7
  [lidar1_intensity] -> Fault Injection Lidar/4
  [camera1_r] -> ROS Send Camera/1
  Fault Injection Lidar/2 -> Lidar Adapter/3
  [gt_camera1_g] -> Fault Injection Camera1/2
  [camera2_g] -> ROS Send Camera 2/2
  Fault Injection Listener Lidar 4/2 -> Fault Injection Lidar3/6
  [fi_lidar_range_variance] -> Fault Injection Listener Lidar 2/2
  CoG offset z/1 -> Car_Pose/9
  [fi_lidar_theta_variance] -> Fault Injection Listener Lidar 4/3
  Fault Injection Lidar3/2 -> Lidar Adapter3/3
  [lidar3_range] -> Fault Injection Lidar2/1
  Fault Injection Listener Camera 2/1 -> Fault Injection Camera/4
  [lidar4_phi] -> Fault Injection Lidar3/3
  Fault Injection Listener Lidar 1/6 -> Fault Injection Lidar/10
  Fault Injection Lidar1/4 -> Lidar Adapter1/5
  Demux1/7 -> Fault Injection Listener TL Camera/8
  Fault Injection Listener Lidar 2/8 -> Fault Injection Lidar1/12
  [lidar3_theta] -> Fault Injection Lidar2/2
  Fault Injection Listener Camera 1/1 -> Fault Injection Camera1/4
  Fault Injection Camera1/3 -> [camera1_b]
  [camera_tl_g] -> ROS Send Camera TL/2
  Camera_1_CM_Demux/3(B) -> [gt_camera1_b], Camera_1_CM_Display/3
  Lidar Adapter2/1 -> [lidar3]
  Demux2/2 -> Fault Injection Listener Camera 2/3
  Fault Injection Listener TL Camera/7 -> Fault Injection Camera2/10
  PointCloudSensor_2_Intensity_Demux/1(Intensity) -> [lidar2_intensity]
  SELF_Demux/6(rotz [deg]) -> [Rotz]
  SELF_Demux/10(velocity [m/s]) -> Dynamics_Empty/1(currant_speed), [velocity]
  SELF_Demux/12(yaw rate [deg/s]) -> [yaw_rate]
  Radar_1_Demux/1(Radar Data) -> [gt_radar]
  PointCloudSensor_1_Intensity_Demux/1(Intensity) -> [lidar1_intensity]
  PointCloudSensor_1_Angles_Demux/2(Phi) -> [lidar1_phi]
  PointCloudSensor_1_Range_Demux/1(Range) -> [lidar1_range]
  PointCloudSensor_1_Angles_Demux/1(Theta) -> [lidar1_theta]
  PointCloudSensor_2_Angles_Demux/2(Phi) -> [lidar2_phi]
  PointCloudSensor_2_Range_Demux/1(Range) -> [lidar2_range]
  PointCloudSensor_2_Angles_Demux/1(Theta) -> [lidar2_theta]
  PointCloudSensor_3_Intensity_Demux/1(Intensity) -> [lidar3_intensity]
  PointCloudSensor_3_Angles_Demux/2(Phi) -> [lidar3_phi]
  PointCloudSensor_3_Angles_Demux/1(Theta) -> [lidar3_theta]
  PointCloudSensor_4_Intensity_Demux/1(Intensity) -> [lidar4_intensity]
  PointCloudSensor_4_Angles_Demux/2(Phi) -> [lidar4_phi]
  PointCloudSensor_4_Range_Demux/1(Range) -> [lidar4_range]
  PointCloudSensor_4_Angles_Demux/1(Theta) -> [lidar4_theta]
  SELF_Demux/2(y [m]) -> [y]
  SELF_Demux/3(z [m]) -> [z]
  SELF_Demux/4(rotx [deg]) -> [Rotx]
  SELF_Demux/5(roty [deg]) -> [Roty]
  PointCloudSensor_3_Range_Demux/1(Range) -> [lidar3_range]
  Dynamics_Empty/1(State) -> STATE_BMW_X5_SUV_1_rc/1
  STATE_BMW_X5_SUV_1_rc/1 -> STATE_BMW_X5_SUV_1_bus/1
  SELF_BMW_X5_SUV_1/1 -> SELF_Demux/1(SELF)
  Radar_1/1 -> Radar_1_Demux/1(Radar)
  PointCloudSensor_1/1 -> PointCloudSensor_1_Range_Demux/1(In1), PointCloudSensor_1_Angles_Demux/1(In2), PointCloudSensor_1_Intensity_Demux/1(In1)
  PointCloudSensor_2/1 -> PointCloudSensor_2_Range_Demux/1(In1), PointCloudSensor_2_Angles_Demux/1(In2), PointCloudSensor_2_Intensity_Demux/1(In1)
  PointCloudSensor_3/1 -> PointCloudSensor_3_Range_Demux/1(In1), PointCloudSensor_3_Angles_Demux/1(In2), PointCloudSensor_3_Intensity_Demux/1(In1)
  PointCloudSensor_4/1 -> PointCloudSensor_4_Range_Demux/1(In1), PointCloudSensor_4_Angles_Demux/1(In2), PointCloudSensor_4_Intensity_Demux/1(In1)
  Camera_1/1 -> Camera_1_CM_Demux/1(In1)
  Camera_tl/1 -> Camera_tl_CM_Demux/1(In1)
  Camera_2/1 -> Camera_2_CM_Demux/1(In1)
  Radar_1_Demux/2(Timestamp) -> Terminator_1/1
  SELF_Demux/7(GPS lat [deg]) -> Terminator_2/1
  SELF_Demux/8(GPS long [deg]) -> Terminator_3/1
  SELF_Demux/9(GPS alt [m]) -> Terminator_4/1
  SELF_Demux/11(heading [deg]) -> Terminator_5/1
  SELF_Demux/13(TimeStamp [s]) -> Terminator_6/1

== system Simulation_cs_old/Camera_1 ==
  Sensor : S-Function  FunctionName=sfun_Camera  Parameters=mbxruntime.parameters.convert(sensorID), mbxruntime.parameters.convert(dataWidth), mbxruntime.parameters.convert(dataHeight), mbxruntime.parameters.convert(channelsPerImage), mbxruntime.parameters.convert(numberOfImages), mbxruntime.parameters.convert(timestep)  SFunctionDeploymentMode=off  EnableBusSupport=off  mask(PreScan Source Block: Camera Sensor){sensorID=163, dataWidth=720, dataHeight=2880, channelsPerImage=3, numberOfImages=1, timestep=1/20}
      mask prompts: sensorID "Sensor ID"; dataWidth "Data width"; dataHeight "Data Height"; channelsPerImage "Channels per image"; numberOfImages "Number of images"; timestep "MATLAB timestep:"
      mask help: The Camera Sensor provides a color or monochrome image.
      mask Help: eval('openHelp(457)')
      mask Display: image(imread('CameraSensor.png'))
  Camera_1 : Outport  Tag=outport/Camera/CameraSensor  OutDataTypeStr=uint8  SampleTime=1/20
  wires:
  Sensor/1 -> Camera_1/1

== system Simulation_cs_old/Camera_2 ==
  Sensor : S-Function  FunctionName=sfun_Camera  Parameters=mbxruntime.parameters.convert(sensorID), mbxruntime.parameters.convert(dataWidth), mbxruntime.parameters.convert(dataHeight), mbxruntime.parameters.convert(channelsPerImage), mbxruntime.parameters.convert(numberOfImages), mbxruntime.parameters.convert(timestep)  SFunctionDeploymentMode=off  EnableBusSupport=off  mask(PreScan Source Block: Camera Sensor){sensorID=166, dataWidth=720, dataHeight=2880, channelsPerImage=3, numberOfImages=1, timestep=1/20}
      mask prompts: sensorID "Sensor ID"; dataWidth "Data width"; dataHeight "Data Height"; channelsPerImage "Channels per image"; numberOfImages "Number of images"; timestep "MATLAB timestep:"
      mask help: The Camera Sensor provides a color or monochrome image.
      mask Help: eval('openHelp(457)')
      mask Display: image(imread('CameraSensor.png'))
  Camera_2 : Outport  Tag=outport/Camera/CameraSensor  OutDataTypeStr=uint8  SampleTime=1/20
  wires:
  Sensor/1 -> Camera_2/1

== system Simulation_cs_old/Camera_tl ==
  Sensor : S-Function  FunctionName=sfun_Camera  Parameters=mbxruntime.parameters.convert(sensorID), mbxruntime.parameters.convert(dataWidth), mbxruntime.parameters.convert(dataHeight), mbxruntime.parameters.convert(channelsPerImage), mbxruntime.parameters.convert(numberOfImages), mbxruntime.parameters.convert(timestep)  SFunctionDeploymentMode=off  EnableBusSupport=off  mask(PreScan Source Block: Camera Sensor){sensorID=164, dataWidth=720, dataHeight=2880, channelsPerImage=3, numberOfImages=1, timestep=1/20}
      mask prompts: sensorID "Sensor ID"; dataWidth "Data width"; dataHeight "Data Height"; channelsPerImage "Channels per image"; numberOfImages "Number of images"; timestep "MATLAB timestep:"
      mask help: The Camera Sensor provides a color or monochrome image.
      mask Help: eval('openHelp(457)')
      mask Display: image(imread('CameraSensor.png'))
  Camera_tl : Outport  Tag=outport/Camera/CameraSensor  OutDataTypeStr=uint8  SampleTime=1/20
  wires:
  Sensor/1 -> Camera_tl/1

== system Simulation_cs_old/Controller ==
  Terminator : Terminator
  sfun_Controller : S-Function  FunctionName=sfun_Controller  Parameters=SParameter1, SParameter2, SParameter3, SParameter4, SParameter5, SParameter6, SParameter7, SParameter8, SParameter9, SParameter10, SampleTime  SFunctionDeploymentMode=off  EnableBusSupport=off  mask(Legacy Function){SFunctionSpec=void prescan_outputFcn(void** work1, PRESCAN_CONTROLLERDATA y1[1]), SParameter1=uint8([ExperimentFile 0]), SParameter2=uint8([ModelDepo 0]), SParameter3=uint8([ControllerOptions 0]), SParameter4=RTmode, SParameter5=PreScanExecutionMode, SParameter6=ControlMode, SParameter7=ControllerCount, SParameter8=ControllerIndex, SParameter9=uint8([SimulationMode 0]), SParameter10=uint8([TargetName 0]), SampleTime=TimeStep, ShowSpec=on}
      mask prompts: SParameter1 "P1:"; SParameter2 "P2:"; SParameter3 "P3:"; SParameter4 "P4:"; SParameter5 "P5:"; SParameter6 "P6:"; SParameter7 "P7:"; SParameter8 "P8:"; SParameter9 "P9:"; SParameter10 "P10:"; SampleTime "Sample time (-1 for inherited):"; ShowSpec "Display function specification"
      mask help:
      | This block allows you to call the legacy functions specified by the following Legacy Code Tool definition:
      | def.SFunctionName = 'sfun_Controller';
      | def.OutputFcnSpec = 'void prescan_outputFcn(void** work1, PRESCAN_CONTROLLERDATA y1[1])';
      | def.StartFcnSpec = 'void prescan_startFcn(void ** work1, uint8 p1[], uint8 p2[], uint8 p3[], double p4, double p5, double p6, double p7, double p8, uint8 p9[], uint8 p10[])';
      | def.TerminateFcnSpec = 'void prescan_terminateFcn(void** work1)';
      | def.HeaderFiles = {'prescan_controller_data.h', 'prescan_SFunLibrary.h', 'prescan_CreateLogHandler.h', 'prescan_CreateErrorHandler.h', 'prescan_modify.h', 'ModuleDLL.h'};
      | def.SourceFiles = {'prescan_MexLogHandler.c', 'prescan_SimStructErrorHandler.c', 'prescan_LogHandler.c', 'prescan_ErrorHandler.c', 'prescan_Modify.c'};
      | def.HostLibFiles = {'sensorinterfaced.lib'};
      | def.TargetLibFiles = {'sensorinterfaced.so'};
      | def.IncPaths = {'.', 'C:\projects\prescan\rt_vislibrary\vis\..\pimp\include\sensors\InterfaceRTW'};
      | def.SrcPaths = {'C:\projects\prescan\rt_vislibrary\vis\..\pimp\include\sensors\InterfaceRTW', 'C:\projects\prescan\rt_vislibrary\vis\..\pimp\include\sensors\InterfaceRTW\ccurrt'};
      | def.LibPaths = {'C:\\projects\\prescan\\vislibrary_build\lib'};
      | def.SampleTime = 'parameterized';
      mask Help: <p>This block was generated automatically by the Legacy Code Tool. For detailed help on this tool, call<a href="matlab:legacy_code('help')"> legacy_code('help')</a>.</p>
      mask Callback ShowSpec:
      | if strcmp(get_param(gcbh, 'ShowSpec'), 'on')
      |   set_param(gcbh, 'MaskDisplay', sprintf('fprintf(''%s'');', get_param(gcbh, 'SFunctionSpec')));
      | else
      |   set_param(gcbh, 'MaskDisplay', sprintf('fprintf(''%s'');', get_param(gcbh, 'FunctionName')));
      | end
      mask Display: fprintf('void prescan_outputFcn(void** work1, PRESCAN_CONTROLLERDATA y1[1])');
  wires:
  sfun_Controller/1 -> Terminator/1
